simulink model "Design_Code"  (R2026a)
settings: Solver=VariableStepAuto
InitFcn:
  | aircraft_inputs;
settings Model: Creator=angee  LastModifiedBy=angee

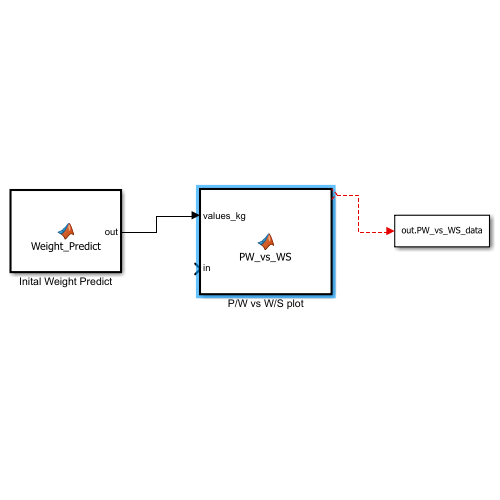
[thumbnail: Simulink's stored preview of the top-level diagram]
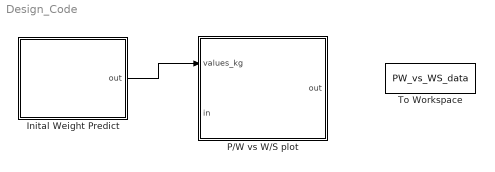
== system Design_Code ==
  Inital Weight Predict : MATLAB Function  TreatAsAtomicUnit=on
  P/W vs W/S plot : MATLAB Function  TreatAsAtomicUnit=on
  To Workspace : ToWorkspace  VariableName=PW_vs_WS_data  SaveFormat=Timeseries  SampleTime=-1
  wires:
  Inital Weight Predict/1(out) -> P/W vs W/S plot/1(values_kg)
  ? -> To Workspace/1

== matlab function Design_Code/P//W vs W//S plot ==
  data: values_kg input; in input; out output
function out = PW_vs_WS(values_kg,in)
% =========================================================================
% SIMULINK COMPATIBLE CONSTRAINT DIAGRAM EVALUATOR BLOCK
% Mirrors AE481_Constraint_Diagram_v9_3.m exactly
% =========================================================================

    g0 = 9.80665;                            % [m/s^2]

    % --- 1. UNPACK WEIGHT RESULTS ---
    m_TO_kg              = values_kg(1);
    m_empty_kg           = values_kg(2);
    m_fuel_kg            = values_kg(3);
    m_crew_pax_kg        = values_kg(4);
    m_baggage_kg         = values_kg(5);
    m_electric_system_kg = values_kg(6);
    m_battery_kg         = values_kg(7);

    W_TO_N = m_TO_kg * g0;                     % takeoff weight force [N]

    range_design_km   = in.range_nmi * 1.852;           
    range_electric_km = in.electricRange_nmi * 1.852;   

    % --- 2. RFP REQUIREMENTS - SI UNITS ---
    Vcruise_threshold_ms = in.Vcruise_threshold_ms;
    Vcruise_objective_ms = in.Vcruise_objective_ms;

    s_TO_req_m = in.s_TO_req_m;
    s_L_req_m  = in.s_L_req_m;

    ROC_RFP_ms = in.ROC_RFP_ms;
    h_obstacle_m = in.h_obstacle_m;

    h_field_m = in.h_field_m;
    dT_field_C = in.dT_field_C;

    h_5000_m = in.h_5000_m;
    dT_5000_C = in.dT_5000_C;

    % --- 3. SELECTED DESIGN ASSUMPTIONS ---
    AR = in.AR;                               
    h_cruise_m = in.h_cruise_m;              
    dT_cruise_C = in.dT_cruise_C;

    beta_cruise  = in.beta_cruise;                     
    beta_landing = in.beta_landing;                     
    beta_climb   = in.beta_climb;   

    CLmax_clean = in.CLmax_clean;
    CLmax_TO    = in.CLmax_TO;
    CLmax_L     = in.CLmax_L;

    wet_c_SI = in.wet_c_SI;
    wet_d    = in.wet_d;
    Cf_equiv = in.Cf_equiv;

    dCD0_TO_flaps = in.dCD0_TO_flaps;    
    dCD0_L_flaps  = in.dCD0_L_flaps;
    dCD0_gear     = in.dCD0_gear;

    e_clean = in.e_clean;       
    e_TO    = in.e_TO;
    e_L     = in.e_L;

    eta_TO     = in.eta_TO;
    eta_climb  = in.eta_climb;
    eta_cruise = in.eta_cruise;
    eta_balked = in.eta_balked;

    powerFrac_TO       = in.powerFrac_TO;
    powerFrac_climb    = in.powerFrac_climb;
    powerFrac_cruise   = in.powerFrac_cruise;
    powerFrac_balked   = in.powerFrac_balked;
    powerFrac_maneuver = in.powerFrac_maneuver;                
    powerFrac_ceiling  = in.powerFrac_ceiling;  

    CLoT_power_remaining = in.CLoT_power_remaining;
    dCD0_CLoT = in.dCD0_CLoT;     
    e_CLoT    = in.e_CLoT;   

    isHighSpeed = in.isHighSpeed; 
    G_initial = in.G_initial;
    G_CLoT = in.G_CLoT;
    G_balked = in.G_balked;

    ks_takeoff = in.ks_takeoff;
    ks_initial = in.ks_initial;
    ks_CLoT    = in.ks_CLoT;
    ks_balked  = in.ks_balked;
    ks_landing = in.ks_landing;

    mu_roll            = in.mu_roll;               
    k_rotation         = in.k_rotation;         
    k_transition       = in.k_transition;       
    gamma_takeoff_deg  = in.gamma_takeoff_deg;                 
    n_transition       = in.n_transition;              

    gamma_approach_deg = in.gamma_approach_deg;
    k_touchdown        = in.k_touchdown;               
    stop_decel_g       = in.stop_decel_g;               
    n_flare            = in.n_flare;              

    battery_specific_energy_Whkg = in.battery_specific_energy_Whkg;
    battery_usable_fraction      = in.battery_usable_fraction;

    eta_battery    = in.eta_battery;
    eta_wiring     = in.eta_wiring;
    eta_controller = in.eta_controller;
    eta_motor      = in.eta_motor;
    eta_prop_elec  = in.eta_prop_elec;

    use_maneuver_constraint = true;
    phi_maneuver_deg  = 60;                   
    n_maneuver        = 1/cosd(phi_maneuver_deg);
    h_maneuver_m      = h_cruise_m;          
    dT_maneuver_C     = dT_cruise_C;
    V_maneuver_ms     = Vcruise_threshold_ms;
    beta_maneuver     = beta_cruise;
    eta_maneuver      = eta_cruise;

    use_ceiling_constraint = true;
    h_ceiling_m       = 12500*0.3048;         
    dT_ceiling_C      = 0;                    
    ROC_ceiling_ms    = 100*0.00508;          
    beta_ceiling      = beta_cruise;          
    eta_ceiling       = eta_cruise;
    ks_ceiling         = 1.10;                

    WS_Nm2 = [linspace(0.1,249.9,500), linspace(250,3000,1000)]; 
    WS_design_fraction = 0.95; 
    PW_design_margin   = 1.05;

    use_stall_constraint = false;             
    Vstall_limit_ms = 50*0.514444;            

    % --- 4. ATMOSPHERE ---
    rho_SL       = atmDensitySI(0,0);
    rho_field    = atmDensitySI(h_field_m,dT_field_C);
    rho_5000     = atmDensitySI(h_5000_m,dT_5000_C);
    rho_cruise   = atmDensitySI(h_cruise_m,dT_cruise_C);
    rho_maneuver = atmDensitySI(h_maneuver_m,dT_maneuver_C);
    rho_ceiling  = atmDensitySI(h_ceiling_m,dT_ceiling_C);

    % --- 5. PARAMETRIC DRAG POLARS ---
    Swet_m2 = 10^(wet_c_SI + wet_d*log10(m_TO_kg));  
    S_grid_m2 = W_TO_N./WS_Nm2;
    f_parasite_m2 = Cf_equiv*Swet_m2;

    CD0_clean = f_parasite_m2./S_grid_m2;
    CD0_TO_GU = CD0_clean + dCD0_TO_flaps;
    CD0_TO_GD = CD0_clean + dCD0_TO_flaps + dCD0_gear;
    CD0_L_GD  = CD0_clean + dCD0_L_flaps  + dCD0_gear;

    % --- 6. W/S LIMITS ---
    sLanding_grid_m = landingDistanceExtremeSTOL_SI( ...
        WS_Nm2,beta_landing,rho_field,CLmax_L,gamma_approach_deg, ...
        k_touchdown,stop_decel_g,h_obstacle_m,n_flare);

    landingOK = sLanding_grid_m <= s_L_req_m;
    if ~any(landingOK)
        WS_landing_max_Nm2 = max(WS_Nm2);
    else
        WS_landing_max_Nm2 = max(WS_Nm2(landingOK));
    end

    if use_stall_constraint
        WS_stall_max_Nm2 = stallWsLimitSI(Vstall_limit_ms,rho_field,CLmax_L,beta_landing);
    else
        WS_stall_max_Nm2 = inf;
    end

    WS_vertical_limit_Nm2 = min(WS_landing_max_Nm2,WS_stall_max_Nm2);

    % --- 7. P/W CONSTRAINTS ---
    K_TO_constraint = 1/(pi*AR*e_TO);
    CL_ground_TO = CLmax_TO/k_rotation^2;
    CD_ground_TO = CD0_TO_GD + K_TO_constraint*CL_ground_TO^2;

    [PW_takeoff_WN,takeoffGeometryOK, ~, ~, ~, ~] = physicsTakeoffPW_SI( ...
        WS_Nm2,s_TO_req_m,h_obstacle_m,rho_field,CLmax_TO, ...
        CL_ground_TO,CD_ground_TO,mu_roll,eta_TO,powerFrac_TO, ...
        k_rotation,k_transition,n_transition,gamma_takeoff_deg);

    PW_RFP_ROC_WN = climbPWfromROC_SI(WS_Nm2,beta_climb,rho_field,eta_climb,CD0_TO_GD,e_TO,AR,CLmax_TO,ks_initial,ROC_RFP_ms,1.0,powerFrac_climb);
    PW_initial_WN = climbPWfromGradient_SI(WS_Nm2,beta_climb,rho_field,eta_climb,CD0_TO_GD,e_TO,AR,CLmax_TO,ks_initial,G_initial,1.0,powerFrac_climb);
    PW_CLoT_WN    = climbPWfromGradient_SI(WS_Nm2,beta_climb,rho_field,eta_climb,CD0_TO_GU+dCD0_CLoT,e_CLoT,AR,CLmax_TO,ks_CLoT,G_CLoT,CLoT_power_remaining,powerFrac_climb);
    PW_balked_WN  = climbPWfromGradient_SI(WS_Nm2,beta_landing,rho_field,eta_balked,CD0_L_GD,e_L,AR,CLmax_L,ks_balked,G_balked,1.0,powerFrac_balked);

    CD0_cruise_ref = 0.018;
    PW_cruise_225_WN = cruisePW_SI(WS_Nm2,beta_cruise,rho_cruise,eta_cruise,CD0_cruise_ref,e_clean,AR,Vcruise_threshold_ms,powerFrac_cruise);

    if use_maneuver_constraint
        [PW_maneuver_WN, maneuverLiftOK] = maneuverPW_SI(WS_Nm2,beta_maneuver,rho_maneuver,eta_maneuver,CD0_cruise_ref,e_clean,AR,CLmax_clean,V_maneuver_ms,n_maneuver,powerFrac_maneuver);
    else
        PW_maneuver_WN = zeros(size(WS_Nm2));
        maneuverLiftOK = true(size(WS_Nm2));
    end

    if use_ceiling_constraint
        [PW_ceiling_WN, ~, ~] = serviceCeilingPW_SI(WS_Nm2,beta_ceiling,rho_ceiling,eta_ceiling,CD0_clean,e_clean,AR,CLmax_clean,ks_ceiling,ROC_ceiling_ms,powerFrac_ceiling);
    else
        PW_ceiling_WN = zeros(size(WS_Nm2));
    end

    % Electric Range Screen
    beta_electric = 1.00;
    V_electric_ms = Vcruise_threshold_ms;
    q_electric = 0.5*rho_cruise*V_electric_ms^2;
    K_electric = 1/(pi*AR*e_clean);

    CL_electric = beta_electric.*WS_Nm2./q_electric;
    CD_electric = CD0_clean + K_electric.*CL_electric.^2;
    D_electric_N = q_electric.*S_grid_m2.*CD_electric;

    eta_electric_total_range = eta_battery*eta_wiring*eta_controller*eta_motor*eta_prop_elec;
    E_battery_usable_J = m_battery_kg*battery_specific_energy_Whkg*3600*battery_usable_fraction;
    E_propulsive_range_J = E_battery_usable_J*eta_electric_total_range;

    R_electric_grid_m = E_propulsive_range_J./D_electric_N;
    R_electric_required_m = range_electric_km*1000;
    electricRangeOK = R_electric_grid_m >= R_electric_required_m;

    % --- 8. FEASIBLE REGION & DESIGN POINT ---
    thresholdMatrix = [PW_takeoff_WN; PW_RFP_ROC_WN; PW_initial_WN; PW_CLoT_WN; PW_balked_WN; PW_cruise_225_WN];
    if use_maneuver_constraint, thresholdMatrix = [thresholdMatrix; PW_maneuver_WN]; end
    if use_ceiling_constraint,  thresholdMatrix = [thresholdMatrix; PW_ceiling_WN]; end

    [PW_envelope_WN,~] = max(thresholdMatrix,[],1);

    verticalOK = WS_Nm2 <= WS_vertical_limit_Nm2;
    combinedFeasible = verticalOK & electricRangeOK & takeoffGeometryOK & maneuverLiftOK;

    if any(combinedFeasible)
        WS_feasible_Nm2 = WS_Nm2(combinedFeasible);
        WS_low_Nm2 = min(WS_feasible_Nm2);
        WS_high_Nm2 = max(WS_feasible_Nm2);
        WS_target_Nm2 = WS_low_Nm2 + WS_design_fraction*(WS_high_Nm2 - WS_low_Nm2);
        [~,iClosestWS] = min(abs(WS_feasible_Nm2 - WS_target_Nm2));
        WS_design_Nm2 = WS_feasible_Nm2(iClosestWS);
        combinedFeasibleExists = true;
    else
        WS_design_Nm2 = WS_design_fraction*WS_vertical_limit_Nm2;
        combinedFeasibleExists = false;
    end

    PW_required_WN = interp1(WS_Nm2,PW_envelope_WN,WS_design_Nm2,'linear','extrap');
    PW_design_WN = PW_design_margin*PW_required_WN;

    S_design_m2 = W_TO_N/WS_design_Nm2;
    P_installed_W  = PW_design_WN*W_TO_N;
    P_installed_kW = P_installed_W/1000;

    mid_idx = round(length(WS_Nm2)/2);
    electricRangePass = double(electricRangeOK(mid_idx));


    out = [WS_design_Nm2, PW_design_WN, S_design_m2, P_installed_kW, electricRangePass]
end

%% ========================================================================
% LOCAL FUNCTIONS - ALL SI
% ========================================================================

function rho = atmDensitySI(h_m,dT_C)
    T0 = 288.15; p0 = 101325; L = 0.0065; g0 = 9.80665; R = 287.05287;
    Tisa = T0 - L*h_m;
    p = p0*(Tisa/T0)^(g0/(R*L));
    Tactual = Tisa + dT_C;
    rho = p/(R*Tactual);
end

function Vstall_ms = stallSpeedSI(WS_TO_Nm2,betaW,rho,CLmax)
    WS_local = betaW*WS_TO_Nm2;
    Vstall_ms = sqrt(2*WS_local/(rho*CLmax));
end

function WSmax_TO_Nm2 = stallWsLimitSI(Vstall_ms,rho,CLmax,betaW)
    WS_condition = 0.5*rho*Vstall_ms^2*CLmax;
    WSmax_TO_Nm2 = WS_condition/betaW;
end

function [PWinstalled_WN,geometryOK,sg_m,str_m,scl_m,htr_m] = physicsTakeoffPW_SI( ...
    WS_Nm2,sTotalReq_m,hObstacle_m,rho,CLmax,CL_TO,CD_TO,mu,etaProp, ...
    powerAvailFrac,kR,kTr,nTransition,gamma_deg)
    g0 = 9.80665;
    gamma = deg2rad(gamma_deg);
    Vs_ms  = sqrt(2.*WS_Nm2./(rho*CLmax));
    Vtr_ms = kTr.*Vs_ms;
    R_m = Vtr_ms.^2./(g0*(nTransition - 1));
    str_full_m = R_m.*sin(gamma);
    htr_full_m = R_m.*(1 - cos(gamma));
    belowObstacle = htr_full_m < hObstacle_m;
    str_m = zeros(size(WS_Nm2)); htr_m = zeros(size(WS_Nm2)); scl_m = zeros(size(WS_Nm2));
    str_m(belowObstacle) = str_full_m(belowObstacle);
    htr_m(belowObstacle) = htr_full_m(belowObstacle);
    scl_m(belowObstacle) = (hObstacle_m - htr_full_m(belowObstacle))./tan(gamma);
    reachesObstacleInTransition = ~belowObstacle;
    if any(reachesObstacleInTransition)
        Rlocal = R_m(reachesObstacleInTransition);
        thetaObs = acos(1 - hObstacle_m./Rlocal);
        str_m(reachesObstacleInTransition) = Rlocal.*sin(thetaObs);
        htr_m(reachesObstacleInTransition) = hObstacle_m;
        scl_m(reachesObstacleInTransition) = 0;
    end
    sg_m = sTotalReq_m - str_m - scl_m;
    geometryOK = sg_m > 0;
    aeroGroundTerm = (kR^2/(2*CLmax)).*(CD_TO - mu*CL_TO);
    TW_required = (kR^2.*WS_Nm2)./(g0*rho*CLmax.*max(sg_m, 1)) + mu + aeroGroundTerm;
    PWavailable_WN = TW_required.*Vtr_ms./etaProp;
    PWinstalled_WN = PWavailable_WN./powerAvailFrac;
    PWinstalled_WN(~geometryOK) = inf;
end

function [sTotal_m,sg_m,str_m,scl_m,htr_m] = physicsTakeoffDistance_SI( ...
    WS_Nm2,PWinstalled_WN,hObstacle_m,rho,CLmax,CL_TO,CD_TO,mu,etaProp, ...
    powerAvailFrac,kR,kTr,nTransition,gamma_deg)
    g0 = 9.80665;
    gamma = deg2rad(gamma_deg);
    Vs_ms  = sqrt(2.*WS_Nm2./(rho*CLmax));
    Vtr_ms = kTr.*Vs_ms;
    PWavailable_WN = PWinstalled_WN.*powerAvailFrac;
    TW_available = etaProp.*PWavailable_WN./Vtr_ms;
    aeroGroundTerm = (kR^2/(2*CLmax)).*(CD_TO - mu*CL_TO);
    accelBracket = TW_available - mu - aeroGroundTerm;
    sg_m = zeros(size(WS_Nm2));
    sg_m(accelBracket > 0) = (kR^2.*WS_Nm2(accelBracket > 0))./(g0*rho*CLmax.*accelBracket(accelBracket > 0));
    sg_m(accelBracket <= 0) = inf;
    R_m = Vtr_ms.^2./(g0*(nTransition - 1));
    str_full_m = R_m.*sin(gamma); htr_full_m = R_m.*(1 - cos(gamma));
    str_m = str_full_m; htr_m = htr_full_m; scl_m = (hObstacle_m - htr_m)./tan(gamma);
    sTotal_m = sg_m + str_m + scl_m;
end

function [sTotal_m, sg_m, sfl_m, sapp_m, hfl_m] = landingDistanceExtremeSTOL_SI( ...
    WS_TO_Nm2, betaW, rho, CLmax, gamma_deg, kTD, decel_g, hObstacle_m, nFlare, safetyFactor)
    if nargin < 9 || isempty(nFlare), nFlare = 1.15; end
    if nargin < 10 || isempty(safetyFactor), safetyFactor = 1.0; end
    g0 = 9.80665; gamma = deg2rad(gamma_deg);
    WS_L_Nm2 = betaW .* WS_TO_Nm2;
    Vs_ms = sqrt(2 .* WS_L_Nm2 ./ (rho * CLmax));
    VTD_ms = kTD .* Vs_ms;
    R_m = VTD_ms.^2 ./ (g0 * (nFlare - 1));
    sfl_full_m = R_m .* sin(gamma); hfl_full_m = R_m .* (1 - cos(gamma));
    belowObstacle = hfl_full_m < hObstacle_m;
    sfl_m = zeros(size(WS_TO_Nm2)); hfl_m = zeros(size(WS_TO_Nm2)); sapp_m = zeros(size(WS_TO_Nm2));
    sfl_m(belowObstacle) = sfl_full_m(belowObstacle);
    hfl_m(belowObstacle) = hfl_full_m(belowObstacle);
    sapp_m(belowObstacle) = (hObstacle_m - hfl_full_m(belowObstacle)) ./ tan(gamma);
    reachesObstacleInFlare = ~belowObstacle;
    if any(reachesObstacleInFlare)
        Rlocal = R_m(reachesObstacleInFlare);
        thetaObs = acos(1 - hObstacle_m ./ Rlocal);
        sfl_m(reachesObstacleInFlare) = Rlocal .* sin(thetaObs);
        hfl_m(reachesObstacleInFlare) = hObstacle_m;
        sapp_m(reachesObstacleInFlare) = 0;
    end
    aStop_ms2 = decel_g * g0;
    sg_m = VTD_ms.^2 ./ (2 * aStop_ms2);
    sTotal_m = (sg_m + sfl_m + sapp_m) .* safetyFactor;
end

function PW_TO_WN = climbPWfromGradient_SI(WS_TO_Nm2,betaW,rho,eta,CD0,e,AR,CLmax,ks,G,powerRemaining,powerAvailFrac)
    WS_local_Nm2 = betaW.*WS_TO_Nm2;
    CL = CLmax/ks^2;
    V_ms = sqrt(2.*WS_local_Nm2./(rho*CL));
    K = 1/(pi*AR*e);
    CD = CD0 + K*CL^2;
    D_over_W = CD./CL;
    PW_current_WN = V_ms./eta .* (D_over_W + G);
    PW_TO_WN = betaW.*PW_current_WN ./ (powerRemaining*powerAvailFrac);
end

function PW_TO_WN = climbPWfromROC_SI(WS_TO_Nm2,betaW,rho,eta,CD0,e,AR,CLmax,ks,ROC_ms,powerRemaining,powerAvailFrac)
    WS_local_Nm2 = betaW.*WS_TO_Nm2;
    CL = CLmax/ks^2;
    V_ms = sqrt(2.*WS_local_Nm2./(rho*CL));
    G = ROC_ms./V_ms;
    PW_TO_WN = climbPWfromGradient_SI(WS_TO_Nm2,betaW,rho,eta,CD0,e,AR,CLmax,ks,G,powerRemaining,powerAvailFrac);
end

function PW_TO_WN = cruisePW_SI(WS_TO_Nm2,betaW,rho,eta,CD0,e,AR,V_ms,powerAvailFrac)
    q_Pa = 0.5*rho*V_ms^2;
    K = 1/(pi*AR*e);
    parasiteTerm = q_Pa*CD0./WS_TO_Nm2;
    inducedTerm = K*betaW^2.*WS_TO_Nm2./q_Pa;
    PW_TO_WN = V_ms/(eta*powerAvailFrac) .* (parasiteTerm + inducedTerm);
end

function [PW_TO_WN,liftOK] = maneuverPW_SI(WS_TO_Nm2,betaW,rho,eta,CD0,e,AR,CLmax,V_ms,n,powerAvailFrac)
    q_Pa = 0.5*rho*V_ms^2;
    WS_maneuver_Nm2 = betaW.*WS_TO_Nm2;
    TW_maneuver = q_Pa.*CD0./WS_maneuver_Nm2 + WS_maneuver_Nm2.*n^2./(q_Pa*pi*AR*e);
    PW_TO_WN = betaW.*TW_maneuver.*V_ms./(eta*powerAvailFrac);
    CL = n.*WS_maneuver_Nm2./q_Pa;
    liftOK = CL <= CLmax;
    PW_TO_WN(~liftOK) = inf;
end

function [PW_TO_WN,Vbest_ms,CLbest] = serviceCeilingPW_SI(WS_TO_Nm2,betaW,rho,eta,CD0,e,AR,CLmax,ksMin,ROC_req_ms,powerAvailFrac)
    K = 1/(pi*AR*e);
    CL_minPower = sqrt(3.*CD0./K);
    CL_stallMargin = CLmax/(ksMin^2);
    CLbest = min(CL_minPower,CL_stallMargin);
    WS_local_Nm2 = betaW.*WS_TO_Nm2;
    Vbest_ms = sqrt(2.*WS_local_Nm2./(rho.*CLbest));
    CD = CD0 + K.*CLbest.^2;
    D_over_W_current = CD./CLbest;
    PW_TO_WN = betaW.*(Vbest_ms.*D_over_W_current + ROC_req_ms) ./ (eta.*powerAvailFrac);
end

== matlab function Design_Code/Inital Weight Predict ==
  data: out output; in parameter
function out = Weight_Predict(in)
%% ========================================================================
%  1. DESIGN INPUTS (Unpacked from input structure)
%  ========================================================================
kgToLb = in.kgToLb;

range_nmi         = in.range_nmi;
cruise_kt         = in.cruise_kt;
altitude_ft       = in.altitude_ft;
LD                = in.LD;
mTO               = in.mTO;
num_people        = in.num_people;
is_electric       = in.is_electric;
electricRange_nmi = in.electricRange_nmi;

climb_kt      = in.climb_kt;
climb_ftmin   = in.climb_ftmin;
descent_kt    = in.descent_kt;
descent_ftmin = in.descent_ftmin;

alternate_nmi = in.alternate_nmi;
reserve_min   = in.reserve_min;

Cp      = in.Cp;
etaProp = in.etaProp;

etaMotor    = in.etaMotor;
etaInverter = in.etaInverter;
etaCable    = in.etaCable;
etaBattery  = in.etaBattery;

pack_Whkg  = in.pack_Whkg;
usableSOC  = in.usableSOC;
pack_kWkg  = in.pack_kWkg;

motor_kWkg    = in.motor_kWkg;
inverter_kWkg = in.inverter_kWkg;

installationFraction = in.installationFraction;

rWarmup  = in.rWarmup;
rTaxi    = in.rTaxi;
rTakeoff = in.rTakeoff;
rClimb   = in.rClimb;
rDescent = in.rDescent;
rLanding = in.rLanding;

% ----- Payload -----
mPeople  = 86.1825 * num_people;                 % Crew + passengers [kg]
mBaggage = 13.6075 * num_people;                 % Baggage [kg]

% ----- Mission -----
prop = logical(is_electric);
if ~prop
    electricRange_nmi = 0;     % Battery-only cruise range [nmi]
end

% ----- Reverse Mission Speed ------
reserve_kt = cruise_kt * 0.8;

% ----- Reserve mission & battery-only contingency -----
if prop == true
    engineOut_nmi        = 20;             % Additional battery-only range [nmi]
    engineOut_kt         = 120;            % Contingency speed [kt]
    electricShaft_kW     = in.electricShaft_kW;
    boost_min            = in.boost_min;
    landing_min          = in.landing_min;
    landingPowerFraction = in.landingPowerFraction;
    auxiliary_kW         = in.auxiliary_kW;
    extraHardware_kg     = 5;
else
    engineOut_nmi        = 0;
    engineOut_kt         = 120;
    electricShaft_kW     = 0;
    boost_min            = 0;
    landing_min          = 0;
    landingPowerFraction = 0;
    auxiliary_kW         = 0;
    extraHardware_kg     = 0;
end

%% ========================================================================
%  2. ELECTRIC PROPULSION ASSUMPTIONS & HARDWARE MASS
%  ========================================================================
etaElectrical = etaMotor * etaInverter * etaCable * etaBattery;
etaOverall = etaProp * etaElectrical;

% Motor mass
mMotor = electricShaft_kW / motor_kWkg;

% Inverter must provide the electrical power entering the motor
inverterPower_kW = electricShaft_kW / etaMotor;
mInverter = inverterPower_kW / inverter_kWkg;

% Installed electric hardware
mElectric = ...
    (mMotor + mInverter) * (1 + installationFraction) ...
    + extraHardware_kg;

%% ========================================================================
%  3. EMPTY-WEIGHT REGRESSION
%  ========================================================================
WTOdata = [1750;
           7255;
           6173;
           8113];
WEdata  = [930;
           4132;
           3075;
           5040];

M = [ones(length(WEdata),1), log10(WEdata)];
R = log10(WTOdata);

coeff = (M.' * M) \ (M.' * R);
A = coeff(1);
B = coeff(2);

%% ========================================================================
%  4. MISSION DISTANCES
%  ========================================================================
climbTime_hr = (altitude_ft / climb_ftmin) / 60;
climbDistance_nmi = climb_kt * climbTime_hr;

descentTime_hr = (altitude_ft / descent_ftmin) / 60;
descentDistance_nmi = descent_kt * descentTime_hr;

fuelCruise_nmi = ...
    range_nmi ...
    - climbDistance_nmi ...
    - descentDistance_nmi ...
    - electricRange_nmi;

assert(electricRange_nmi >= 0, ...
    'Electric range cannot be negative.');
assert(fuelCruise_nmi >= 0, ...
    'Fuel cruise range cannot be negative');

%% ========================================================================
%  5. FUEL FRACTION
%  ========================================================================
K_Breguet = 325.9; % Converts customary units to nmi

reserveEquivalent_nmi = reserve_kt * reserve_min / 60;

fuelPoweredRange_nmi = ...
    fuelCruise_nmi ...
    + alternate_nmi ...
    + reserveEquivalent_nmi;

rFuelCruise = exp( ...
    -fuelPoweredRange_nmi * Cp ...
    / (K_Breguet * etaProp * LD) );

missionWeightRatio = ...
    rWarmup ...
    * rTaxi ...
    * rTakeoff ...
    * rClimb ...
    * rFuelCruise ...
    * rDescent ...
    * rLanding;

fuelFraction = 1 - missionWeightRatio;

%% ========================================================================
%  6. FIXED-POINT TAKEOFF-WEIGHT ITERATION
%  ========================================================================
tolerance     = 1e-6;
maxIterations = 5000;
converged     = false;

for iteration = 1:maxIterations
    WTO_lb = mTO * kgToLb;
    WEconventional_lb = ...
        10^((log10(WTO_lb) - A) / B);
    mConventional = WEconventional_lb / kgToLb;
    
    mEmpty = mConventional + mElectric;
    mFuel = fuelFraction * mTO;

    Eflight_kWh = ...
        mTO * 9.80665 ...
        * (electricRange_nmi + engineOut_nmi) * 1852 ...
        / (LD * etaOverall * 3.6e6);

    Eboost_kWh = ...
        (electricShaft_kW / etaElectrical) ...
        * boost_min / 60;

    Elanding_kWh = ...
        (electricShaft_kW * landingPowerFraction ...
        / etaElectrical) * landing_min / 60;

    electricHours = ...
        (boost_min + landing_min) / 60 ...
        + electricRange_nmi / cruise_kt ...
        + engineOut_nmi / engineOut_kt;
        
    Eaux_kWh = ...
        (auxiliary_kW / etaBattery) ...
        * electricHours;

    Erequired_kWh = ...
        Eflight_kWh ...
        + Eboost_kWh ...
        + Elanding_kWh ...
        + Eaux_kWh;

    mBatteryEnergy = ...
        1000 * Erequired_kWh ...
        / (pack_Whkg * usableSOC);

    batteryChemicalPower_kW = ...
        electricShaft_kW / etaElectrical ...
        + auxiliary_kW / etaBattery;
        
    mBatteryPower = ...
        batteryChemicalPower_kW / pack_kWkg;

    mBattery = max( ...
        mBatteryEnergy, ...
        mBatteryPower );

    mTO_new = ...
        mEmpty ...
        + mFuel ...
        + mPeople ...
        + mBaggage ...
        + mBattery;

    relativeError = ...
        abs(mTO_new - mTO) / mTO_new;
    mTO = mTO_new;

    if relativeError < tolerance
        converged = true;
        break;
    end
    
    assert( ...
        isfinite(mTO) && mTO > 0 && mTO < 25000, ...
        ['No weight closure within the numerical search limit. ' ...
         'Revisit the design assumptions.'] );
end

assert( ...
    converged, ...
    'Weight iteration did not converge.' );

%% ========================================================================
%  7. WEIGHTS - NUMERIC OUTPUT VECTOR
%  ========================================================================
values_kg = [ ...
    mTO, ...
    mEmpty, ...
    mFuel, ...
    mPeople, ...
    mBaggage, ...
    mElectric, ...
    mBattery ];

%% ========================================================================
%  8. BOOKKEEPING CHECK
%  ========================================================================
massCheck = ...
    mEmpty ...
    + mFuel ...
    + mPeople ...
    + mBaggage ...
    + mBattery;

assert( ...
    abs(massCheck - mTO) < 1e-3, ...
    'Final weight bookkeeping does not balance.' );

% Output the clean numeric vector to Simulink
out = values_kg;
end
